simulink model "Benchmark_model"  (R2018a)
settings: Solver=ode1  StartTime=0  StopTime=t_end  FixedStep=simTs  RelTol=1e-3  EnableMultiTasking=on
values from neighbouring files (symbols this model uses):
  driv_rect_time = 0.5    [Initial_parameters.m]
  gamma = 25    [Initial_parameters.m]
  hw_min = 3    [Initial_parameters.m]
  Initial_eng_spd = 0    [Initial_parameters.m]
  Initial_headway = Sensor_FOL_dDist(2)    [Initial_parameters.m]
  Initial_SOC = 50    [Initial_parameters.m]
  Initial_vhcl_spd = 0    [Initial_parameters.m]
  spd_lim = 60    [Initial_parameters.m]
undefined symbols (not defined in the file or in its folder): Route_Distance, Route_Slope
(part 1 of 2)
settings Model: PauseTimes=100  Creator=1562880  LastModifiedBy=Lenovo
settings DataIOCC: SaveFormat=Structure  SaveOutput=off  SignalLogging=off  DSMLogging=off  SaveTime=off
settings OptimizationCC: BooleanDataType=off  DefaultParameterBehavior=Inlined  LifeSpan=1
settings DebuggingCC: SolverPrmCheckMsg=warning  FcnCallInpInsideContextMsg=warning  StateNameClashWarn=warning  SFUnexpectedBacktrackingDiag=warning  SFNoUnconditionalDefaultTransitionDiag=warning  SFExecutionAtInitializationDiag=none
settings CodeAppCC: StateflowObjectComments=on
settings GRTTargetCC: TargetLangStandard=C89/C90 (ANSI)  GeneratePreprocessorConditionals=Disable all
settings ConfigComp: CovMetricSettings=dw  CovHtmlReporting=on  CovSaveCumulativeToWorkspaceVar=on  CovSaveSingleToWorkspaceVar=on  CovExternalEMLEnable=off

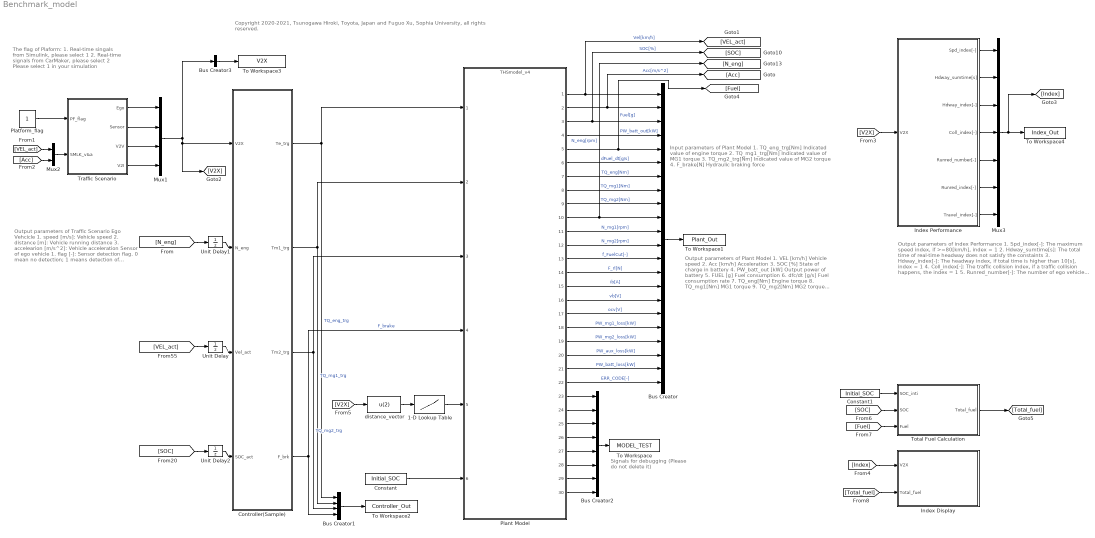
== system Benchmark_model ==
  note: The flag of Plaform:
      |
      | 1. Real-time singals from Simulink, please select 1
      | 2. Real-time signals from CarMaker, please select 2
      | Please select 1 in your simulation
  note: Signals for debugging
      | (Please do not delete it)
  note: Input parameters of Plant Model
      |
      | 1. TQ_eng_trg[Nm] Indicated value of engine torque
      | 2. TQ_mg1_trg[Nm] Indicated value of MG1 torque
      | 3. TQ_mg2_trg[Nm] Indicated value of MG2 torque
      | 4. F_brake[N] Hydraulic braking force
  note: Output parameters of Plant Model
      |
      | 1. VEL [km/h] Vehicle speed
      | 2. Acc [km/h] Acceleration
      | 3. SOC [%] State of charge in battery
      | 4. PW_batt_out [kW] Output power of battery
      | 5. FUEL [g] Fuel consumption
      | 6. dfc/dt [g/s] Fuel consumption rate
      |
      | 7. TQ_eng[Nm] Engine torque
      | 8. TQ_mg1[Nm] MG1 torque
      | 9. TQ_mg2[Nm] MG2 torque
      |
      | 10. N_eng[rpm] Engine speed
      | 11. N_mg1[rpm] MG1 speed
      | 12. N_mg2[rpm] MG2 speed
      |
      | 13. f_FuelCut[-] FuelCut flag
      | 14. F_rl [N] Resistance
      | 15. ib[A] Battery current
      | 16. vb[V] Battery voltage
      | 17. ocv[V] Open circuit voltage
      |
      | 18. PW_mg1_loss[kW] MG1 electricity loss
      | 19. PW_mg2_loss[kW] MG2 electricity loss
      |
      | 20. PW_aux_loss[kW] Auxiliary loss
      | 21. PW_batt_loss[kW] Battery electricity loss
      |
      | 22. ERR_CODE Error code
  note: Copyright 2020-2021, Tsunogawa Hiroki, Toyota, Japan and Fuguo Xu, Sophia University, all rights reserved.
  note: Output parameters of Traffic Scenario
      |
      | Ego Vehcicle
      | 1. speed [m/s]: Vehicle speed
      | 2. distance [m]: Vehicle running distance
      | 3. accelearion [m/s^2]: Vehicle acceleration
      |
      | Sensor of ego vehicle
      | 1. flag [-]: Sensor detection flag. 0 mean no detection; 1 means detection of preceding vehicle. When Platform_flag = 1, detection flag is 'nan', no signal from Simulink.
      | 2. dist headway [m]: distance headway, when flag=0, it is 0
      |
      | V2V information
      | 1. pre_speed [m/s]: Preceding vehicle speed
      | 2. pre_diastance [m]: Preceding vehicle running distance
      | 3. pre_acceleration [m/s^2]: Preceding vehicle acceleration
      |
      | V2I information
      | 1.state_next_1st [-]: the phase of 1st next traffic light
      | 2. tRemain_next_1st [s]: the remaining time of 1st next traffic light
      | 3. s2inters_next_1st [m]: distance to the 1st next intersection
      | 4. state_next_2nd [-]: the phase of 2nd next traffic light
      | 5. tRemain_next_2nd [s]: the remaining time of 2nd next traffic light
      | 6. s2inters_next_2st [m]: distance to the 2nd next intersection
  note: Output parameters of index Performance
      |
      | 1. Spd_index[-]: The maximum speed index, if >=80[km/h], index = 1
      |
      | 2. Hdway_sumtime[s]: The total time of real-time headway does not satisfy the constaints
      | 3. Hdway_index[-]: The headway index, if total time is higher than 10[s], index = 1
      |
      | 4. Coll_index[-]: The traffic collision index, if a traffic collision happens, the index = 1
      |
      | 5. Runred_number[-]: The number of ego vehicle runs a red light
      | 6. Runred_index[-]: The run red index, if the total number is higher than 2, index = 1
      | 7. Travel_index[-]: When the toal travel time of ego vehicle is higher than time of pre vhcl plus 30 [sec], index = 1
  " Index Display" : Subsystem
  " Index Performance" : Subsystem
  1-D Lookup Table : Lookup_n-D  NumberOfTableDimensions=1  BreakpointsForDimension1=Route_Distance  Table=Route_Slope  InternalRulePriority=Speed  RndMeth=Simplest  InputSameDT=on
  Bus Creator : BusCreator  Inputs=22
  Bus Creator1 : BusCreator  Inputs=4
  Bus Creator2 : BusCreator  Inputs=8
  Bus Creator3 : BusCreator  Inputs=1
  Constant : Constant  Value=Initial_SOC
  Constant1 : Constant  Value=Initial_SOC
  Controller(Sample) : Subsystem
  Mux1 : Mux
  Mux2 : Mux  Inputs=2
  Mux3 : Mux  Inputs=7
  Plant Model : ModelReference  ModelNameDialog=THSmodel_v4.slxp  ModelReferenceVersion=1.632  CopyOfModelProtected=on
  Platform_flag : Constant
  To Workspace : ToWorkspace  VariableName=MODEL_TEST  SaveFormat=Timeseries  SampleTime=-1
  To Workspace1 : ToWorkspace  VariableName=Plant_Out  SaveFormat=Timeseries  SampleTime=-1
  To Workspace2 : ToWorkspace  VariableName=Controller_Out  SaveFormat=Timeseries  SampleTime=-1
  To Workspace3 : ToWorkspace  VariableName=V2X  SaveFormat=Timeseries  SampleTime=-1
  To Workspace4 : ToWorkspace  VariableName=Index_Out  SaveFormat=Timeseries  SampleTime=-1
  Total Fuel Calculation : Subsystem
  Traffic Scenario : Subsystem
  Unit Delay : UnitDelay  InitialCondition=Initial_vhcl_spd  SampleTime=-1
  Unit Delay1 : UnitDelay  InitialCondition=Initial_eng_spd  SampleTime=-1
  Unit Delay2 : UnitDelay  InitialCondition=Initial_SOC  SampleTime=-1
  distance_vector : Fcn  Expr=u(2)
  wires:
  Plant Model/1 -> Bus Creator/1, [VEL_act]  "Vel[km/h]"
  Plant Model/2 -> Bus Creator/2, [Acc]  "Acc[m/s^2]"
  Plant Model/3 -> Bus Creator/3, [SOC]  "SOC[%]"
  Plant Model/11 -> Bus Creator/11  "N_mg1[rpm]"
  Plant Model/10 -> Bus Creator/10, [N_eng]  "N_eng[rpm]"
  Plant Model/4 -> Bus Creator/4  "PW_batt_out[kW]"
  Plant Model/5 -> [Fuel], Bus Creator/5  "Fuel[g]"
  Plant Model/9 -> Bus Creator/9  "TQ_mg2[Nm]"
  Plant Model/8 -> Bus Creator/8  "TQ_mg1[Nm]"
  Plant Model/6 -> Bus Creator/6  "dFuel_dt[g/s]"
  Plant Model/7 -> Bus Creator/7  "TQ_eng[Nm]"
  Plant Model/12 -> Bus Creator/12  "N_mg2[rpm]"
  Plant Model/13 -> Bus Creator/13  "f_FuelCut[-]"
  Plant Model/14 -> Bus Creator/14  "F_rl[N]"
  Plant Model/15 -> Bus Creator/15  "ib[A]"
  Plant Model/16 -> Bus Creator/16  "vb[V]"
  Plant Model/17 -> Bus Creator/17  "ocv[V]"
  Plant Model/25 -> Bus Creator2/3
  Plant Model/23 -> Bus Creator2/1
  Plant Model/24 -> Bus Creator2/2
  Controller(Sample)/4(F_brk) -> Plant Model/4, Bus Creator1/4  "F_brake"
  Controller(Sample)/2(Tm1_trg) -> Plant Model/2, Bus Creator1/2  "TQ_mg1_trg"
  Controller(Sample)/1(Te_trg) -> Plant Model/1, Bus Creator1/1  "TQ_eng_trg"
  Controller(Sample)/3(Tm2_trg) -> Plant Model/3, Bus Creator1/3  "TQ_mg2_trg"
  [N_eng] -> Unit Delay1/1
  [VEL_act] -> Unit Delay/1
  Unit Delay/1 -> Controller(Sample)/3(Vel_act)
  Unit Delay1/1 -> Controller(Sample)/2(N_eng)
  [SOC] -> Unit Delay2/1
  Unit Delay2/1 -> Controller(Sample)/4(SOC_act)
  Plant Model/18 -> Bus Creator/18  "PW_mg1_loss[kW]"
  Plant Model/19 -> Bus Creator/19  "PW_mg2_loss[kW]"
  Plant Model/22 -> Bus Creator/22  "ERR_CODE[-]"
  Plant Model/20 -> Bus Creator/20  "PW_aux_loss[kW]"
  Plant Model/21 -> Bus Creator/21  "PW_batt_loss[kW]"
  Plant Model/26 -> Bus Creator2/4
  Plant Model/27 -> Bus Creator2/5
  Plant Model/28 -> Bus Creator2/6
  Plant Model/29 -> Bus Creator2/7
  Plant Model/30 -> Bus Creator2/8
  Bus Creator/1 -> To Workspace1/1
  Bus Creator1/1 -> To Workspace2/1
  Bus Creator2/1 -> To Workspace/1
  Bus Creator3/1 -> To Workspace3/1
  Mux1/1 -> Controller(Sample)/1(V2X), [V2X], Bus Creator3/1
  Mux2/1 -> Traffic Scenario/2(SMLK_v&a)
  [Acc] -> Mux2/2
  [VEL_act] -> Mux2/1
  Platform_flag/1 -> Traffic Scenario/1(PF_flag)
  Traffic Scenario/1(Ego) -> Mux1/1
  Traffic Scenario/2(Sensor) -> Mux1/2
  Traffic Scenario/3(V2V) -> Mux1/3
  Traffic Scenario/4(V2I) -> Mux1/4
  [V2X] -> " Index Performance"/1(V2X)
  Mux3/1 -> [Index], To Workspace4/1
  [Index] -> " Index Display"/1(V2X)
  " Index Performance"/1(Spd_index[-]) -> Mux3/1
  " Index Performance"/2(Hdway_sumtime[s]) -> Mux3/2
  " Index Performance"/3(Hdway_index[-]) -> Mux3/3
  " Index Performance"/4(Coll_index[-]) -> Mux3/4
  " Index Performance"/5(Runred_number[-]) -> Mux3/5
  " Index Performance"/6(Runred_index[-]) -> Mux3/6
  distance_vector/1 -> 1-D Lookup Table/1
  Constant/1 -> Plant Model/6
  1-D Lookup Table/1 -> Plant Model/5
  [V2X] -> distance_vector/1
  [SOC] -> Total Fuel Calculation/2(SOC)
  [Fuel] -> Total Fuel Calculation/3(Fuel)
  Constant1/1 -> Total Fuel Calculation/1(SOC_inti)
  Total Fuel Calculation/1(Total_fuel) -> [Total_fuel]
  [Total_fuel] -> " Index Display"/2(Total_fuel)
  " Index Performance"/7(Travel_index[-]) -> Mux3/7

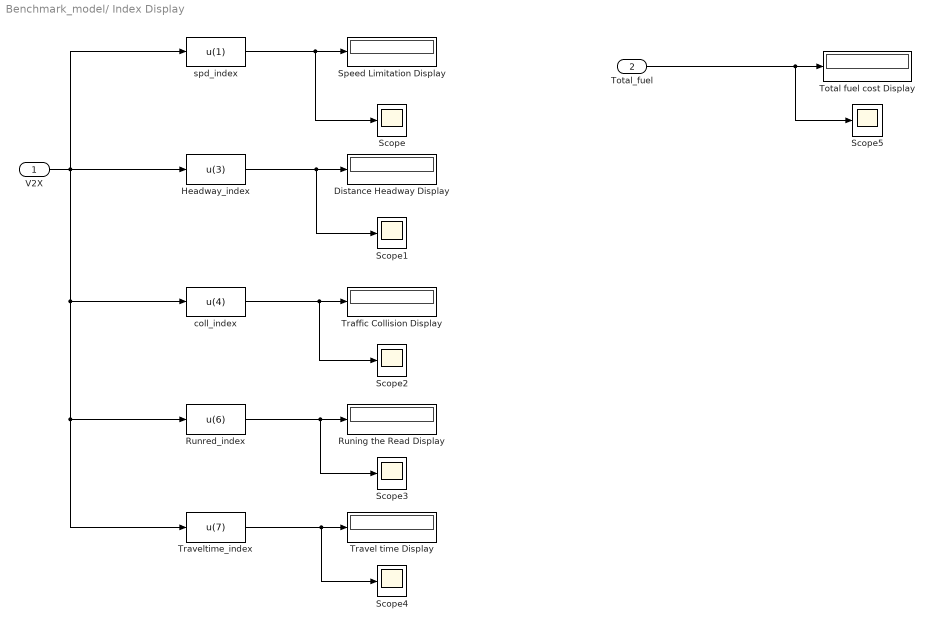
== system Benchmark_model/ Index Display ==
  V2X : Inport
  Total_fuel : Inport  Port=2
  Distance Headway Display : Display
  Headway_index : Fcn  Expr=u(3)
  Runing the Read Display : Display
  Runred_index : Fcn  Expr=u(6)
  Scope{,1..5} (6 alike) : Scope
  Speed Limitation Display : Display
  Total fuel cost Display : Display
  Traffic Collision Display : Display
  Travel time Display : Display
  Traveltime_index : Fcn  Expr=u(7)
  coll_index : Fcn  Expr=u(4)
  spd_index : Fcn  Expr=u(1)
  wires:
  V2X/1 -> spd_index/1, Headway_index/1, Traveltime_index/1, Runred_index/1, coll_index/1
  spd_index/1 -> Scope/1, Speed Limitation Display/1
  coll_index/1 -> Scope2/1, Traffic Collision Display/1
  Headway_index/1 -> Scope1/1, Distance Headway Display/1
  Runred_index/1 -> Scope3/1, Runing the Read Display/1
  Traveltime_index/1 -> Scope4/1, Travel time Display/1
  Total_fuel/1 -> Scope5/1, Total fuel cost Display/1

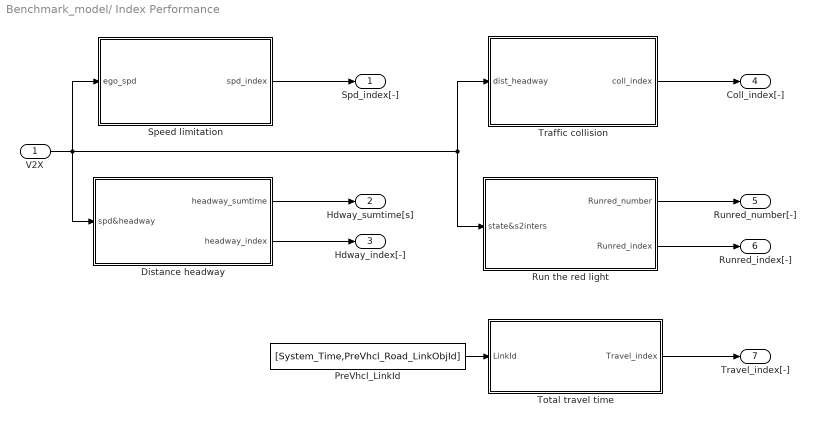
== system Benchmark_model/ Index Performance ==
  V2X : Inport
  Distance headway : Subsystem
  PreVhcl_LinkId : FromWorkspace  VariableName=[System_Time,PreVhcl_Road_LinkObjId]  SampleTime=0
  Run the red light : Subsystem
  Speed limitation : Subsystem
  Total travel time : Subsystem
  Traffic collision : Subsystem
  Spd_index[-] : Outport
  Hdway_sumtime[s] : Outport  Port=2
  Hdway_index[-] : Outport  Port=3
  Coll_index[-] : Outport  Port=4
  Runred_number[-] : Outport  Port=5
  Runred_index[-] : Outport  Port=6
  Travel_index[-] : Outport  Port=7
  wires:
  V2X/1 -> Distance headway/1(spd&headway), Traffic collision/1(dist_headway), Run the red light/1(state&s2inters), Speed limitation/1(ego_spd)
  Traffic collision/1(coll_index) -> Coll_index[-]/1
  Speed limitation/1(spd_index) -> Spd_index[-]/1
  Distance headway/1(headway_sumtime) -> Hdway_sumtime[s]/1
  Distance headway/2(headway_index) -> Hdway_index[-]/1
  Run the red light/2(Runred_index) -> Runred_index[-]/1
  Run the red light/1(Runred_number) -> Runred_number[-]/1
  PreVhcl_LinkId/1 -> Total travel time/1(LinkId)
  Total travel time/1(Travel_index) -> Travel_index[-]/1

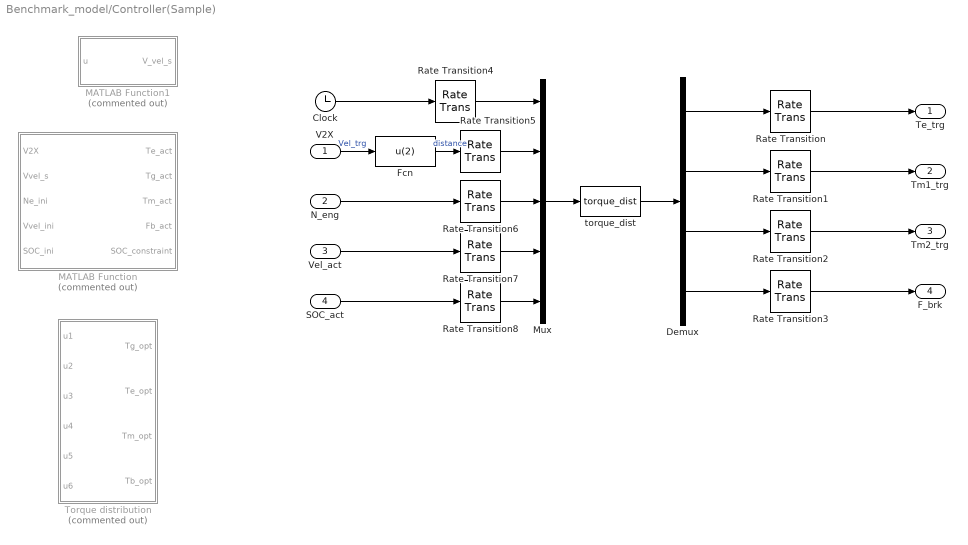
== system Benchmark_model/Controller(Sample) ==
  V2X : Inport
  N_eng : Inport  Port=2
  Vel_act : Inport  Port=3
  SOC_act : Inport  Port=4
  Clock : Clock
      settings: Decimation=50
  Demux : Demux
  Fcn : Fcn  Expr=u(2)
  MATLAB Function : MATLAB Function  Commented=on  TreatAsAtomicUnit=on
  MATLAB Function1 : MATLAB Function  Commented=on  TreatAsAtomicUnit=on
  Mux : Mux  Inputs=5
  Rate Transition{,1..3} (4 alike) : RateTransition  OutPortSampleTime=0.01
  Rate Transition{4..8} (5 alike) : RateTransition  OutPortSampleTime=0.05
  Torque distribution : MATLAB Function  Commented=on  TreatAsAtomicUnit=on
  torque_dist : MATLABFcn  MATLABFcn=torque_dist  OutputDimensions=4  SampleTime=0.05
  Te_trg : Outport
  Tm1_trg : Outport  Port=2
  Tm2_trg : Outport  Port=3
  F_brk : Outport  Port=4
  wires:
  Demux/1 -> Rate Transition/1
  Demux/2 -> Rate Transition1/1
  Demux/3 -> Rate Transition2/1
  Demux/4 -> Rate Transition3/1
  V2X/1 -> Fcn/1  "Vel_trg"
  N_eng/1 -> Rate Transition6/1
  Vel_act/1 -> Rate Transition7/1
  SOC_act/1 -> Rate Transition8/1
  Clock/1 -> Rate Transition4/1
  Fcn/1 -> Rate Transition5/1  "distance"
  Rate Transition/1 -> Te_trg/1
  Rate Transition1/1 -> Tm1_trg/1
  Rate Transition2/1 -> Tm2_trg/1
  Rate Transition3/1 -> F_brk/1
  Mux/1 -> torque_dist/1
  torque_dist/1 -> Demux/1
  Rate Transition4/1 -> Mux/1
  Rate Transition5/1 -> Mux/2
  Rate Transition8/1 -> Mux/5
  Rate Transition7/1 -> Mux/4
  Rate Transition6/1 -> Mux/3

== system Benchmark_model/Total Fuel Calculation ==
  SOC_inti : Inport
  SOC : Inport  Port=2
  Fuel : Inport  Port=3
  Add : Sum
  Add1 : Sum  Inputs=+-
  equivalent factor : Gain  Gain=gamma
  Total_fuel : Outport
  wires:
  SOC/1 -> Add1/2
  Fuel/1 -> Add/2
  equivalent factor/1 -> Add/1
  Add/1 -> Total_fuel/1
  SOC_inti/1 -> Add1/1
  Add1/1 -> equivalent factor/1

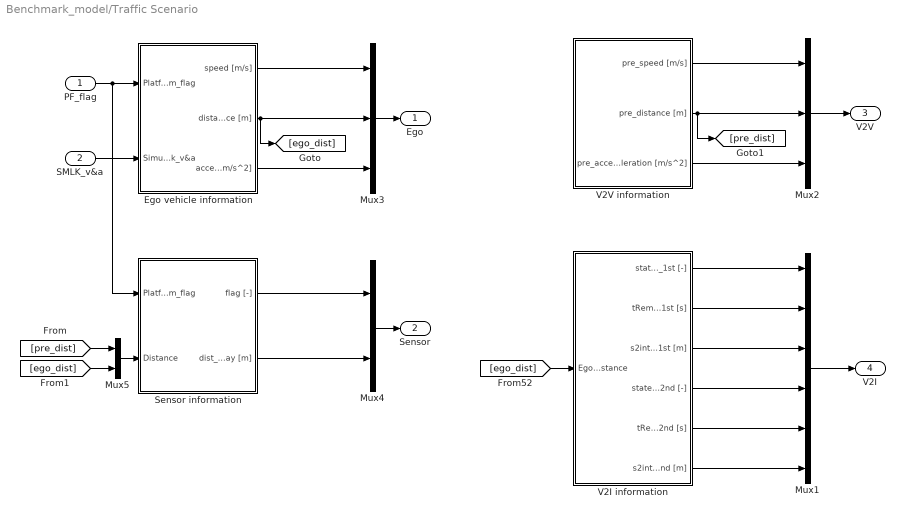
== system Benchmark_model/Traffic Scenario ==
  PF_flag : Inport
  SMLK_v&a : Inport  Port=2
  "Ego vehicle information " : Subsystem
  Mux1 : Mux  Inputs=6
  Mux2 : Mux  Inputs=3
  Mux3 : Mux  Inputs=3
  Mux4 : Mux  Inputs=2
  Mux5 : Mux  Inputs=2
  Sensor information : Subsystem
  V2I information : Subsystem
  V2V information : Subsystem
  Ego : Outport
  Sensor : Outport  Port=2
  V2V : Outport  Port=3
  V2I : Outport  Port=4
  wires:
  [ego_dist] -> V2I information/1(Ego_distance)
  "Ego vehicle information "/2(distance [m]) -> Mux3/2, [ego_dist]
  V2I information/1(state_next_1st [-]) -> Mux1/1
  V2I information/2(tRemain_next_1st [s]) -> Mux1/2
  Mux1/1 -> V2I/1
  Mux2/1 -> V2V/1
  V2V information/1(pre_speed [m/s]) -> Mux2/1
  V2V information/2(pre_distance [m]) -> [pre_dist], Mux2/2
  V2V information/3(pre_acceleration [m/s^2]) -> Mux2/3
  "Ego vehicle information "/1(speed [m/s]) -> Mux3/1
  "Ego vehicle information "/3(acceleration [m/s^2]) -> Mux3/3
  Mux3/1 -> Ego/1
  Sensor information/1(flag [-]) -> Mux4/1
  Mux4/1 -> Sensor/1
  PF_flag/1 -> Sensor information/1(Platform_flag), "Ego vehicle information "/1(Platform_flag)
  SMLK_v&a/1 -> "Ego vehicle information "/2(Simulink_v&a)
  Mux5/1 -> Sensor information/2(Distance)
  [ego_dist] -> Mux5/2
  [pre_dist] -> Mux5/1
  Sensor information/2(dist_headway [m]) -> Mux4/2
  V2I information/3(s2inters_next_1st [m]) -> Mux1/3
  V2I information/4(state_next_2nd [-]) -> Mux1/4
  V2I information/5(tRemain_next_2nd [s]) -> Mux1/5
  V2I information/6(s2inters_next_2nd [m]) -> Mux1/6

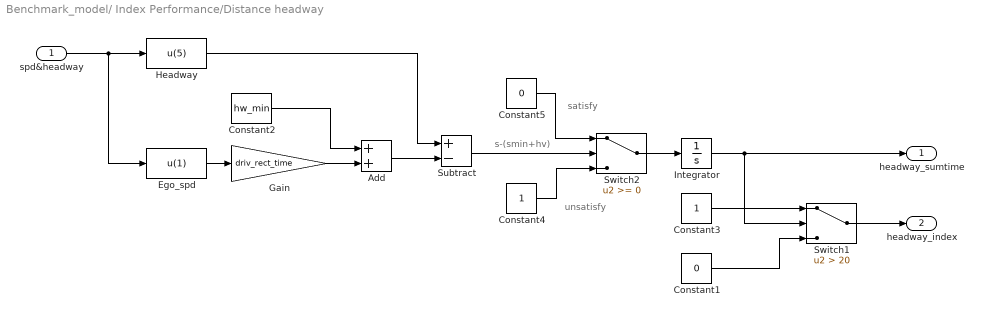
== system Benchmark_model/ Index Performance/Distance headway ==
  note: unsatisfy
  note: satisfy
  note: s-(smin+hv)
  spd&headway : Inport
  Add : Sum
  Constant1 : Constant  Value=0
  Constant2 : Constant  Value=hw_min
  Constant3 : Constant
  Constant4 : Constant
  Constant5 : Constant  Value=0
  Ego_spd : Fcn  Expr=u(1)
  Gain : Gain  Gain=driv_rect_time
  Headway : Fcn  Expr=u(5)
  Integrator : Integrator
  Subtract : Sum  Inputs=+-
  Switch1 : Switch  Criteria=u2 > Threshold  Threshold=20
  Switch2 : Switch
  headway_sumtime : Outport
  headway_index : Outport  Port=2
  wires:
  spd&headway/1 -> Headway/1, Ego_spd/1
  Ego_spd/1 -> Gain/1
  Gain/1 -> Add/2
  Constant2/1 -> Add/1
  Add/1 -> Subtract/2
  Headway/1 -> Subtract/1
  Switch2/1 -> Integrator/1
  Integrator/1 -> Switch1/2, headway_sumtime/1
  Constant1/1 -> Switch1/3
  Constant3/1 -> Switch1/1
  Switch1/1 -> headway_index/1
  Constant4/1 -> Switch2/3
  Constant5/1 -> Switch2/1
  Subtract/1 -> Switch2/2

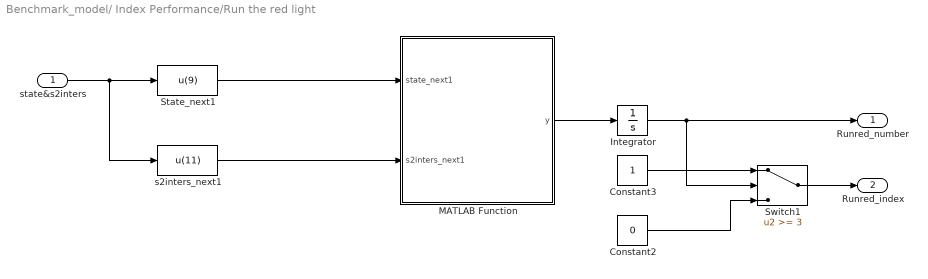
== system Benchmark_model/ Index Performance/Run the red light ==
  state&s2inters : Inport
  Constant2 : Constant  Value=0
  Constant3 : Constant
  Integrator : Integrator
  MATLAB Function : MATLAB Function  TreatAsAtomicUnit=on
  State_next1 : Fcn  Expr=u(9)
  Switch1 : Switch  Threshold=3
  s2inters_next1 : Fcn  Expr=u(11)
  Runred_number : Outport
  Runred_index : Outport  Port=2
  wires:
  MATLAB Function/1(y) -> Integrator/1
  state&s2inters/1 -> s2inters_next1/1, State_next1/1
  s2inters_next1/1 -> MATLAB Function/2(s2inters_next1)
  State_next1/1 -> MATLAB Function/1(state_next1)
  Integrator/1 -> Switch1/2, Runred_number/1
  Constant2/1 -> Switch1/3
  Constant3/1 -> Switch1/1
  Switch1/1 -> Runred_index/1

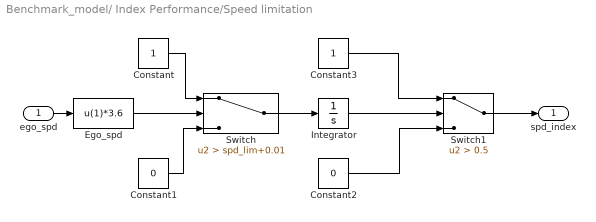
== system Benchmark_model/ Index Performance/Speed limitation ==
  ego_spd : Inport
  Constant : Constant
  Constant1 : Constant  Value=0
  Constant2 : Constant  Value=0
  Constant3 : Constant
  Ego_spd : Fcn  Expr=u(1)*3.6
  Integrator : Integrator
  Switch : Switch  Criteria=u2 > Threshold  Threshold=spd_lim+0.01
  Switch1 : Switch  Criteria=u2 > Threshold  Threshold=0.5
  spd_index : Outport
  wires:
  Constant/1 -> Switch/1
  Constant1/1 -> Switch/3
  Ego_spd/1 -> Switch/2
  ego_spd/1 -> Ego_spd/1
  Switch1/1 -> spd_index/1
  Integrator/1 -> Switch1/2
  Constant3/1 -> Switch1/1
  Constant2/1 -> Switch1/3
  Switch/1 -> Integrator/1

== system Benchmark_model/ Index Performance/Total travel time ==
  LinkId : Inport
  Clock : Clock
  Constant : Constant
  Constant1 : Constant  Value=0
  MATLAB Function : MATLAB Function  TreatAsAtomicUnit=on
  Subtract : Sum  Inputs=-+
  Switch : Switch  Criteria=u2 > Threshold  Threshold=60*2+30
  Travel_index : Outport
  wires:
  Constant1/1 -> Switch/3
  Clock/1 -> Subtract/2, MATLAB Function/2(Sys_time)
  Constant/1 -> Switch/1
  Subtract/1 -> Switch/2
  Switch/1 -> Travel_index/1
  MATLAB Function/1(pre_terminal_time) -> Subtract/1
  LinkId/1 -> MATLAB Function/1(LinkId)

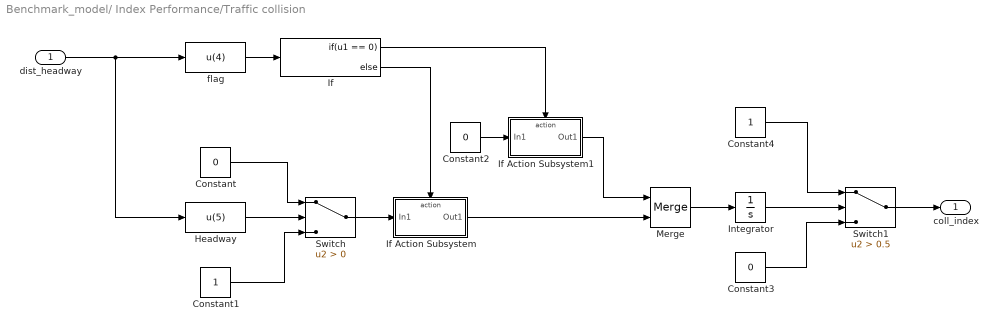
== system Benchmark_model/ Index Performance/Traffic collision ==
  dist_headway : Inport
  Constant : Constant  Value=0
  Constant1 : Constant
  Constant2 : Constant  Value=0
  Constant3 : Constant  Value=0
  Constant4 : Constant
  Headway : Fcn  Expr=u(5)
  If : If  IfExpression=u1 == 0
  If Action Subsystem : Subsystem  TreatAsAtomicUnit=on
  If Action Subsystem1 : Subsystem  TreatAsAtomicUnit=on
  Integrator : Integrator
  Merge : Merge
  Switch : Switch  Criteria=u2 > Threshold
  Switch1 : Switch  Criteria=u2 > Threshold  Threshold=0.5
  flag : Fcn  Expr=u(4)
  coll_index : Outport
  wires:
  dist_headway/1 -> Headway/1, flag/1
  Headway/1 -> Switch/2
  Constant/1 -> Switch/1
  Constant1/1 -> Switch/3
  flag/1 -> If/1
  If/2 -> If Action Subsystem/Action
  If/1 -> If Action Subsystem1/Action
  If Action Subsystem1/1(Out1) -> Merge/1
  If Action Subsystem/1(Out1) -> Merge/2
  Constant2/1 -> If Action Subsystem1/1(In1)
  Switch/1 -> If Action Subsystem/1(In1)
  Integrator/1 -> Switch1/2
  Constant4/1 -> Switch1/1
  Constant3/1 -> Switch1/3
  Switch1/1 -> coll_index/1
  Merge/1 -> Integrator/1

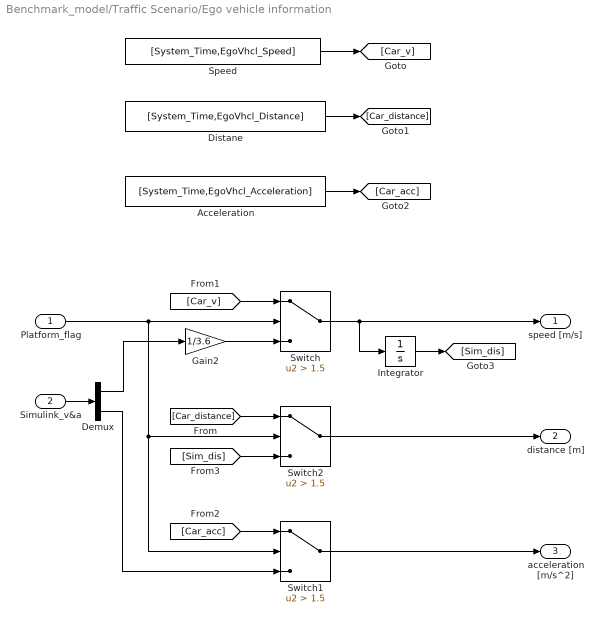
== system Benchmark_model/Traffic Scenario/Ego vehicle information  ==
  Platform_flag : Inport
  Simulink_v&a : Inport  Port=2
  Acceleration : FromWorkspace  VariableName=[System_Time,EgoVhcl_Acceleration]  SampleTime=0
  Demux : Demux  Outputs=2
  Distane : FromWorkspace  VariableName=[System_Time,EgoVhcl_Distance]  SampleTime=0
  Gain2 : Gain  Gain=1/3.6
  Integrator : Integrator
  Speed : FromWorkspace  VariableName=[System_Time,EgoVhcl_Speed]  SampleTime=0
  Switch : Switch  Criteria=u2 > Threshold  Threshold=1.5
  Switch1 : Switch  Criteria=u2 > Threshold  Threshold=1.5
  Switch2 : Switch  Criteria=u2 > Threshold  Threshold=1.5
  speed [m/s] : Outport
  distance [m] : Outport  Port=2
  acceleration [m/s^2] : Outport  Port=3
  wires:
  Platform_flag/1 -> Switch/2, Switch2/2, Switch1/2
  Simulink_v&a/1 -> Demux/1
  Demux/1 -> Gain2/1
  Demux/2 -> Switch1/3
  Switch/1 -> Integrator/1, speed [m/s]/1
  Speed/1 -> [Car_v]
  Distane/1 -> [Car_distance]
  Acceleration/1 -> [Car_acc]
  [Car_v] -> Switch/1
  [Car_acc] -> Switch1/1
  [Car_distance] -> Switch2/1
  Integrator/1 -> [Sim_dis]
  [Sim_dis] -> Switch2/3
  Switch1/1 -> acceleration [m/s^2]/1
  Switch2/1 -> distance [m]/1
  Gain2/1 -> Switch/3

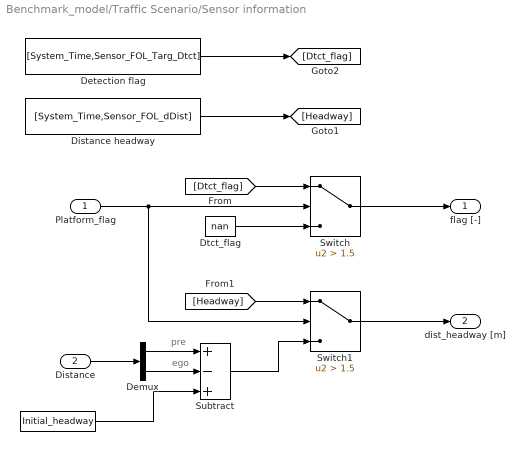
== system Benchmark_model/Traffic Scenario/Sensor information ==
  note: ego
  note: pre
  Platform_flag : Inport
  Distance : Inport  Port=2
  " " : Constant  Value=Initial_headway
  Demux : Demux  Outputs=2
  Detection flag : FromWorkspace  VariableName=[System_Time,Sensor_FOL_Targ_Dtct]  SampleTime=0
  Distance headway : FromWorkspace  VariableName=[System_Time,Sensor_FOL_dDist]  SampleTime=0
  Dtct_flag : Constant  Value=nan
  Subtract : Sum  Inputs=+-+
  Switch : Switch  Criteria=u2 > Threshold  Threshold=1.5
  Switch1 : Switch  Criteria=u2 > Threshold  Threshold=1.5
  flag [-] : Outport
  dist_headway [m] : Outport  Port=2
  wires:
  Platform_flag/1 -> Switch1/2, Switch/2
  Detection flag/1 -> [Dtct_flag]
  Distance headway/1 -> [Headway]
  [Headway] -> Switch1/1
  Switch/1 -> flag [-]/1
  [Dtct_flag] -> Switch/1
  Dtct_flag/1 -> Switch/3
  Switch1/1 -> dist_headway [m]/1
  Distance/1 -> Demux/1
  Subtract/1 -> Switch1/3
  Demux/1 -> Subtract/1
  Demux/2 -> Subtract/2
  " "/1 -> Subtract/3

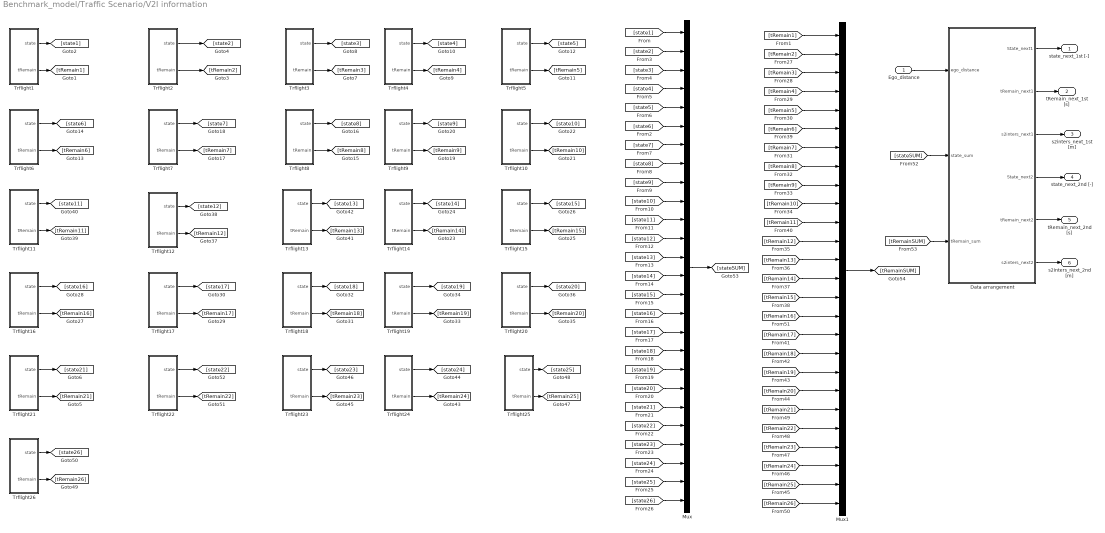
== system Benchmark_model/Traffic Scenario/V2I information ==
  Ego_distance : Inport
  Data arrangement : MATLAB Function  TreatAsAtomicUnit=on
  Mux : Mux  Inputs=26
  Mux1 : Mux  Inputs=26
  Trflight1 : Subsystem
  Trflight10 : Subsystem
  Trflight11 : Subsystem
  Trflight12 : Subsystem
  Trflight13 : Subsystem
  Trflight14 : Subsystem
  Trflight15 : Subsystem
  Trflight16 : Subsystem
  Trflight17 : Subsystem
  Trflight18 : Subsystem
  Trflight19 : Subsystem
  Trflight2 : Subsystem
  Trflight20 : Subsystem
  Trflight21 : Subsystem
  Trflight22 : Subsystem
  Trflight23 : Subsystem
  Trflight24 : Subsystem
  Trflight25 : Subsystem
  Trflight26 : Subsystem
  Trflight3 : Subsystem
  Trflight4 : Subsystem
  Trflight5 : Subsystem
  Trflight6 : Subsystem
  Trflight7 : Subsystem
  Trflight8 : Subsystem
  Trflight9 : Subsystem
  state_next_1st [-] : Outport
  tRemain_next_1st [s] : Outport  Port=2
  s2inters_next_1st [m] : Outport  Port=3
  state_next_2nd [-] : Outport  Port=4
  tRemain_next_2nd [s] : Outport  Port=5
  s2inters_next_2nd [m] : Outport  Port=6
  wires:
  Trflight26/1(state) -> [state26]
  Trflight2/2(tRemain) -> [tRemain2]
  Trflight2/1(state) -> [state2]
  Trflight26/2(tRemain) -> [tRemain26]
  Trflight1/1(state) -> [state1]
  Trflight1/2(tRemain) -> [tRemain1]
  Trflight3/2(tRemain) -> [tRemain3]
  Trflight3/1(state) -> [state3]
  Trflight4/2(tRemain) -> [tRemain4]
  Trflight4/1(state) -> [state4]
  Trflight5/2(tRemain) -> [tRemain5]
  Trflight5/1(state) -> [state5]
  Trflight6/1(state) -> [state6]
  Trflight6/2(tRemain) -> [tRemain6]
  Trflight7/1(state) -> [state7]
  Trflight7/2(tRemain) -> [tRemain7]
  Trflight8/1(state) -> [state8]
  Trflight8/2(tRemain) -> [tRemain8]
  Trflight9/1(state) -> [state9]
  Trflight9/2(tRemain) -> [tRemain9]
  Trflight10/1(state) -> [state10]
  Trflight10/2(tRemain) -> [tRemain10]
  Trflight16/1(state) -> [state16]
  Trflight16/2(tRemain) -> [tRemain16]
  Trflight17/1(state) -> [state17]
  Trflight17/2(tRemain) -> [tRemain17]
  Trflight18/1(state) -> [state18]
  Trflight18/2(tRemain) -> [tRemain18]
  Trflight19/1(state) -> [state19]
  Trflight19/2(tRemain) -> [tRemain19]
  Trflight20/1(state) -> [state20]
  Trflight20/2(tRemain) -> [tRemain20]
  Trflight15/1(state) -> [state15]
  Trflight15/2(tRemain) -> [tRemain15]
  Trflight14/1(state) -> [state14]
  Trflight14/2(tRemain) -> [tRemain14]
  Trflight13/1(state) -> [state13]
  Trflight13/2(tRemain) -> [tRemain13]
  Trflight12/1(state) -> [state12]
  Trflight12/2(tRemain) -> [tRemain12]
  Trflight11/2(tRemain) -> [tRemain11]
  Trflight11/1(state) -> [state11]
  Trflight21/1(state) -> [state21]
  Trflight21/2(tRemain) -> [tRemain21]
  Trflight22/1(state) -> [state22]
  Trflight22/2(tRemain) -> [tRemain22]
  Trflight23/1(state) -> [state23]
  Trflight23/2(tRemain) -> [tRemain23]
  Trflight24/1(state) -> [state24]
  Trflight24/2(tRemain) -> [tRemain24]
  Trflight25/1(state) -> [state25]
  Trflight25/2(tRemain) -> [tRemain25]
  [state1] -> Mux/1
  [state3] -> Mux/3
  [state2] -> Mux/2
  [state5] -> Mux/5
  [state6] -> Mux/6
  [state7] -> Mux/7
  [state8] -> Mux/8
  [state9] -> Mux/9
  [state4] -> Mux/4
  [state10] -> Mux/10
  [state11] -> Mux/11
  [state12] -> Mux/12
  [state13] -> Mux/13
  [state14] -> Mux/14
  [state15] -> Mux/15
  [state16] -> Mux/16
  [state17] -> Mux/17
  [state18] -> Mux/18
  [state19] -> Mux/19
  [state20] -> Mux/20
  [state26] -> Mux/26
  [state21] -> Mux/21
  [state22] -> Mux/22
  [state23] -> Mux/23
  [state24] -> Mux/24
  [state25] -> Mux/25
  [tRemain3] -> Mux1/3
  [tRemain2] -> Mux1/2
  [tRemain1] -> Mux1/1
  [tRemain4] -> Mux1/4
  [tRemain5] -> Mux1/5
  [tRemain6] -> Mux1/6
  [tRemain7] -> Mux1/7
  [tRemain8] -> Mux1/8
  [tRemain9] -> Mux1/9
  [tRemain10] -> Mux1/10
  [tRemain11] -> Mux1/11
  [tRemain12] -> Mux1/12
  [tRemain15] -> Mux1/15
  [tRemain14] -> Mux1/14
  [tRemain13] -> Mux1/13
  [tRemain16] -> Mux1/16
  [tRemain26] -> Mux1/26
  [tRemain18] -> Mux1/18
  [tRemain17] -> Mux1/17
  [tRemain21] -> Mux1/21
  [tRemain20] -> Mux1/20
  [tRemain19] -> Mux1/19
  [tRemain25] -> Mux1/25
  [tRemain24] -> Mux1/24
  [tRemain23] -> Mux1/23
  [tRemain22] -> Mux1/22
  Mux/1 -> [stateSUM]
  Mux1/1 -> [tRemainSUM]
  Data arrangement/1(State_next1) -> state_next_1st [-]/1
  Data arrangement/2(tRemain_next1) -> tRemain_next_1st [s]/1
  Data arrangement/4(State_next2) -> state_next_2nd [-]/1
  Data arrangement/5(tRemain_next2) -> tRemain_next_2nd [s]/1
  [stateSUM] -> Data arrangement/2(state_sum)
  [tRemainSUM] -> Data arrangement/3(tRemain_sum)
  Ego_distance/1 -> Data arrangement/1(ego_distance)
  Data arrangement/3(s2inters_next1) -> s2inters_next_1st [m]/1
  Data arrangement/6(s2inters_next2) -> s2inters_next_2nd [m]/1

== system Benchmark_model/Traffic Scenario/V2V information ==
  Preceding vehicle acceleration : FromWorkspace  VariableName=[System_Time,PreVhcl_Acceleration]  SampleTime=0
  Preceding vehicle distance : FromWorkspace  VariableName=[System_Time,PreVhcl_Distance]  SampleTime=0
  Preceding vehicle speed : FromWorkspace  VariableName=[System_Time,PreVhcl_Speed]  SampleTime=0
  pre_speed [m/s] : Outport
  pre_distance [m] : Outport  Port=2
  pre_acceleration [m/s^2] : Outport  Port=3
  wires:
  Preceding vehicle distance/1 -> pre_distance [m]/1
  Preceding vehicle acceleration/1 -> pre_acceleration [m/s^2]/1
  Preceding vehicle speed/1 -> pre_speed [m/s]/1

== system Benchmark_model/ Index Performance/Traffic collision/If Action Subsystem ==
  In1 : Inport
  Action Port : ActionPort  ActionType=else
  Out1 : Outport
  wires:
  In1/1 -> Out1/1

== system Benchmark_model/ Index Performance/Traffic collision/If Action Subsystem1 ==
  In1 : Inport
  Action Port : ActionPort  ActionType=then
  Out1 : Outport
  wires:
  In1/1 -> Out1/1

== system Benchmark_model/Traffic Scenario/V2I information/Trflight1 ==
  Traffic light state : FromWorkspace  VariableName=[System_Time,TrfLight_State_TL1]  SampleTime=0
  Traffic light tRemain : FromWorkspace  VariableName=[System_Time,TrfLight_tRemain_TL1]  SampleTime=0
  state : Outport
  tRemain : Outport  Port=2
  wires:
  Traffic light state/1 -> state/1
  Traffic light tRemain/1 -> tRemain/1

== system Benchmark_model/Traffic Scenario/V2I information/Trflight10 ==
  Traffic light state : FromWorkspace  VariableName=[System_Time,TrfLight_State_TL10]  SampleTime=0
  Traffic light tRemain : FromWorkspace  VariableName=[System_Time,TrfLight_tRemain_TL10]  SampleTime=0
  state : Outport
  tRemain : Outport  Port=2
  wires:
  Traffic light tRemain/1 -> tRemain/1
  Traffic light state/1 -> state/1

== system Benchmark_model/Traffic Scenario/V2I information/Trflight11 ==
  Traffic light state : FromWorkspace  VariableName=[System_Time,TrfLight_State_TL11]  SampleTime=0
  Traffic light tRemain : FromWorkspace  VariableName=[System_Time,TrfLight_tRemain_TL11]  SampleTime=0
  state : Outport
  tRemain : Outport  Port=2
  wires:
  Traffic light state/1 -> state/1
  Traffic light tRemain/1 -> tRemain/1

== system Benchmark_model/Traffic Scenario/V2I information/Trflight12 ==
  Traffic light state : FromWorkspace  VariableName=[System_Time,TrfLight_State_TL12]  SampleTime=0
  Traffic light tRemain : FromWorkspace  VariableName=[System_Time,TrfLight_tRemain_TL12]  SampleTime=0
  state : Outport
  tRemain : Outport  Port=2
  wires:
  Traffic light tRemain/1 -> tRemain/1
  Traffic light state/1 -> state/1

== system Benchmark_model/Traffic Scenario/V2I information/Trflight13 ==
  Traffic light state : FromWorkspace  VariableName=[System_Time,TrfLight_State_TL13]  SampleTime=0
  Traffic light tRemain : FromWorkspace  VariableName=[System_Time,TrfLight_tRemain_TL13]  SampleTime=0
  state : Outport
  tRemain : Outport  Port=2
  wires:
  Traffic light tRemain/1 -> tRemain/1
  Traffic light state/1 -> state/1

== system Benchmark_model/Traffic Scenario/V2I information/Trflight14 ==
  Traffic light state : FromWorkspace  VariableName=[System_Time,TrfLight_State_TL14]  SampleTime=0
  Traffic light tRemain : FromWorkspace  VariableName=[System_Time,TrfLight_tRemain_TL14]  SampleTime=0
  state : Outport
  tRemain : Outport  Port=2
  wires:
  Traffic light state/1 -> state/1
  Traffic light tRemain/1 -> tRemain/1

== system Benchmark_model/Traffic Scenario/V2I information/Trflight15 ==
  Traffic light state : FromWorkspace  VariableName=[System_Time,TrfLight_State_TL15]  SampleTime=0
  Traffic light tRemain : FromWorkspace  VariableName=[System_Time,TrfLight_tRemain_TL15]  SampleTime=0
  state : Outport
  tRemain : Outport  Port=2
  wires:
  Traffic light tRemain/1 -> tRemain/1
  Traffic light state/1 -> state/1

== system Benchmark_model/Traffic Scenario/V2I information/Trflight16 ==
  Traffic light state : FromWorkspace  VariableName=[System_Time,TrfLight_State_TL16]  SampleTime=0
  Traffic light tRemain : FromWorkspace  VariableName=[System_Time,TrfLight_tRemain_TL16]  SampleTime=0
  state : Outport
  tRemain : Outport  Port=2
  wires:
  Traffic light state/1 -> state/1
  Traffic light tRemain/1 -> tRemain/1

== system Benchmark_model/Traffic Scenario/V2I information/Trflight17 ==
  Traffic light state : FromWorkspace  VariableName=[System_Time,TrfLight_State_TL17]  SampleTime=0
  Traffic light tRemain : FromWorkspace  VariableName=[System_Time,TrfLight_tRemain_TL17]  SampleTime=0
  state : Outport
  tRemain : Outport  Port=2
  wires:
  Traffic light tRemain/1 -> tRemain/1
  Traffic light state/1 -> state/1

== system Benchmark_model/Traffic Scenario/V2I information/Trflight18 ==
  Traffic light state : FromWorkspace  VariableName=[System_Time,TrfLight_State_TL18]  SampleTime=0
  Traffic light tRemain : FromWorkspace  VariableName=[System_Time,TrfLight_tRemain_TL18]  SampleTime=0
  state : Outport
  tRemain : Outport  Port=2
  wires:
  Traffic light state/1 -> state/1
  Traffic light tRemain/1 -> tRemain/1

== system Benchmark_model/Traffic Scenario/V2I information/Trflight19 ==
  Traffic light state : FromWorkspace  VariableName=[System_Time,TrfLight_State_TL19]  SampleTime=0
  Traffic light tRemain : FromWorkspace  VariableName=[System_Time,TrfLight_tRemain_TL19]  SampleTime=0
  state : Outport
  tRemain : Outport  Port=2
  wires:
  Traffic light tRemain/1 -> tRemain/1
  Traffic light state/1 -> state/1

== system Benchmark_model/Traffic Scenario/V2I information/Trflight2 ==
  Traffic light state : FromWorkspace  VariableName=[System_Time,TrfLight_State_TL2]  SampleTime=0
  Traffic light tRemain : FromWorkspace  VariableName=[System_Time,TrfLight_tRemain_TL2]  SampleTime=0
  state : Outport
  tRemain : Outport  Port=2
  wires:
  Traffic light tRemain/1 -> tRemain/1
  Traffic light state/1 -> state/1

== system Benchmark_model/Traffic Scenario/V2I information/Trflight20 ==
  Traffic light state : FromWorkspace  VariableName=[System_Time,TrfLight_State_TL20]  SampleTime=0
  Traffic light tRemain : FromWorkspace  VariableName=[System_Time,TrfLight_tRemain_TL20]  SampleTime=0
  state : Outport
  tRemain : Outport  Port=2
  wires:
  Traffic light state/1 -> state/1
  Traffic light tRemain/1 -> tRemain/1

== system Benchmark_model/Traffic Scenario/V2I information/Trflight21 ==
  Traffic light state : FromWorkspace  VariableName=[System_Time,TrfLight_State_TL21]  SampleTime=0
  Traffic light tRemain : FromWorkspace  VariableName=[System_Time,TrfLight_tRemain_TL21]  SampleTime=0
  state : Outport
  tRemain : Outport  Port=2
  wires:
  Traffic light state/1 -> state/1
  Traffic light tRemain/1 -> tRemain/1

== system Benchmark_model/Traffic Scenario/V2I information/Trflight22 ==
  Traffic light state : FromWorkspace  VariableName=[System_Time,TrfLight_State_TL22]  SampleTime=0
  Traffic light tRemain : FromWorkspace  VariableName=[System_Time,TrfLight_tRemain_TL22]  SampleTime=0
  state : Outport
  tRemain : Outport  Port=2
  wires:
  Traffic light tRemain/1 -> tRemain/1
  Traffic light state/1 -> state/1

== system Benchmark_model/Traffic Scenario/V2I information/Trflight23 ==
  Traffic light state : FromWorkspace  VariableName=[System_Time,TrfLight_State_TL23]  SampleTime=0
  Traffic light tRemain : FromWorkspace  VariableName=[System_Time,TrfLight_tRemain_TL23]  SampleTime=0
  state : Outport
  tRemain : Outport  Port=2
  wires:
  Traffic light state/1 -> state/1
  Traffic light tRemain/1 -> tRemain/1

== system Benchmark_model/Traffic Scenario/V2I information/Trflight24 ==
  Traffic light state : FromWorkspace  VariableName=[System_Time,TrfLight_State_TL24]  SampleTime=0
  Traffic light tRemain : FromWorkspace  VariableName=[System_Time,TrfLight_tRemain_TL24]  SampleTime=0
  state : Outport
  tRemain : Outport  Port=2
  wires:
  Traffic light tRemain/1 -> tRemain/1
  Traffic light state/1 -> state/1

== system Benchmark_model/Traffic Scenario/V2I information/Trflight25 ==
  Traffic light state : FromWorkspace  VariableName=[System_Time,TrfLight_State_TL25]  SampleTime=0
  Traffic light tRemain : FromWorkspace  VariableName=[System_Time,TrfLight_tRemain_TL25]  SampleTime=0
  state : Outport
  tRemain : Outport  Port=2
  wires:
  Traffic light state/1 -> state/1
  Traffic light tRemain/1 -> tRemain/1

== system Benchmark_model/Traffic Scenario/V2I information/Trflight26 ==
  Traffic light state : FromWorkspace  VariableName=[System_Time,TrfLight_State_TL26]  SampleTime=0
  Traffic light tRemain : FromWorkspace  VariableName=[System_Time,TrfLight_tRemain_TL26]  SampleTime=0
  state : Outport
  tRemain : Outport  Port=2
  wires:
  Traffic light tRemain/1 -> tRemain/1
  Traffic light state/1 -> state/1

== system Benchmark_model/Traffic Scenario/V2I information/Trflight3 ==
  Traffic light state : FromWorkspace  VariableName=[System_Time,TrfLight_State_TL3]  SampleTime=0
  Traffic light tRemain : FromWorkspace  VariableName=[System_Time,TrfLight_tRemain_TL3]  SampleTime=0
  state : Outport
  tRemain : Outport  Port=2
  wires:
  Traffic light state/1 -> state/1
  Traffic light tRemain/1 -> tRemain/1

== system Benchmark_model/Traffic Scenario/V2I information/Trflight4 ==
  Traffic light state : FromWorkspace  VariableName=[System_Time,TrfLight_State_TL4]  SampleTime=0
  Traffic light tRemain : FromWorkspace  VariableName=[System_Time,TrfLight_tRemain_TL4]  SampleTime=0
  state : Outport
  tRemain : Outport  Port=2
  wires:
  Traffic light tRemain/1 -> tRemain/1
  Traffic light state/1 -> state/1

== system Benchmark_model/Traffic Scenario/V2I information/Trflight5 ==
  Traffic light state : FromWorkspace  VariableName=[System_Time,TrfLight_State_TL5]  SampleTime=0
  Traffic light tRemain : FromWorkspace  VariableName=[System_Time,TrfLight_tRemain_TL5]  SampleTime=0
  state : Outport
  tRemain : Outport  Port=2
  wires:
  Traffic light state/1 -> state/1
  Traffic light tRemain/1 -> tRemain/1

== system Benchmark_model/Traffic Scenario/V2I information/Trflight6 ==
  Traffic light state : FromWorkspace  VariableName=[System_Time,TrfLight_State_TL6]  SampleTime=0
  Traffic light tRemain : FromWorkspace  VariableName=[System_Time,TrfLight_tRemain_TL6]  SampleTime=0
  state : Outport
  tRemain : Outport  Port=2
  wires:
  Traffic light tRemain/1 -> tRemain/1
  Traffic light state/1 -> state/1

== system Benchmark_model/Traffic Scenario/V2I information/Trflight7 ==
  Traffic light state : FromWorkspace  VariableName=[System_Time,TrfLight_State_TL7]  SampleTime=0
  Traffic light tRemain : FromWorkspace  VariableName=[System_Time,TrfLight_tRemain_TL7]  SampleTime=0
  state : Outport
  tRemain : Outport  Port=2
  wires:
  Traffic light state/1 -> state/1
  Traffic light tRemain/1 -> tRemain/1

== system Benchmark_model/Traffic Scenario/V2I information/Trflight8 ==
  Traffic light state : FromWorkspace  VariableName=[System_Time,TrfLight_State_TL8]  SampleTime=0
  Traffic light tRemain : FromWorkspace  VariableName=[System_Time,TrfLight_tRemain_TL8]  SampleTime=0
  state : Outport
  tRemain : Outport  Port=2
  wires:
  Traffic light tRemain/1 -> tRemain/1
  Traffic light state/1 -> state/1

== system Benchmark_model/Traffic Scenario/V2I information/Trflight9 ==
  Traffic light state : FromWorkspace  VariableName=[System_Time,TrfLight_State_TL9]  SampleTime=0
  Traffic light tRemain : FromWorkspace  VariableName=[System_Time,TrfLight_tRemain_TL9]  SampleTime=0
  state : Outport
  tRemain : Outport  Port=2
  wires:
  Traffic light state/1 -> state/1
  Traffic light tRemain/1 -> tRemain/1

== matlab function Benchmark_model/ Index Performance/Total travel time/MATLAB Function ==
  settings: updateMethod=DISCRETE
  data: LinkId input; pre_terminal_time output; Sys_time input
function pre_terminal_time = fcn(LinkId,Sys_time)
persistent Sys_time_stop index_time
if isempty(Sys_time_stop)
    Sys_time_stop = 0;
    index_time = 0;
end

error_index = (index_time==0)&&(LinkId==2215);
if  error_index == 1
    index_time = 1;
    Sys_time_stop = Sys_time;
else                             % distance to stop line<19 and previous distance>=15, red light
    if index_time == 0
    Sys_time_stop = Sys_time;
    end
end

pre_terminal_time = Sys_time_stop;
